simulink model "youBot_Arm_before_acceleration_test"  (R2024a)
settings: Solver=ode15s  StartTime=0.0  StopTime=3.3  MaxStep=1e-2  RelTol=1e-3  AbsTol=1e-4
model workspace: external: MATLAB File youBot_DataFile.m (data not in the file)
undefined symbols (not defined in the file): Extr_Data_LinkHoles, Qt, sigbuilder_block, smiData, X, Y, YBT_Par, Z
libraries: sm_lib x193, nesl_utility x130, fl_lib x53, simulink x13, Parts_Lib x10, MyMath_lib x8, Motor_Lib x5, Contact_Forces_Lib x4, ee_lib x2, sdl_lib x2
(part 6 of 8)

== system youBot_Arm_before_acceleration_test/Arm/Actuation/Motor/Gripper/Motor ==
  C : Inport
  Meas P : Subsystem  Tag=CustomStyle
      mask Display: disp('m')
  Motor : Motor_Lib/Motor  VariantControl=Motor  r_motor=YBT_Par.Gripper.Motor.R  l_motor=YBT_Par.Gripper.Motor.L  k_motor=1/YBT_Par.Gripper.Motor.K  i_motor_noLoad=YBT_Par.Gripper.Motor.no_load_i  v_supply=YBT_Par.Battery.v  gear_ratio=YBT_Par.Gripper.Motor.gr  friction_visc=YBT_Par.Gripper.Motor.friction  ctrl_deadZone=YBT_Par.Control.Dead_Band
  RevoluteWristGripperPivot : sm_lib/Joints/Revolute Joint  JointMode=Normal  CompositeWrenchDir=FollowerOnBase  CompositeWrenchFrame=BaseFrame  SenseConstraintForce=on  SenseConstraintTorque=off  SenseTotalForce=off  SenseTotalTorque=off  PositionTargetSpecify=on  PositionTargetPriority=Low  PositionTargetValue=smiData.RevoluteJoint(4).Rz.Pos  PositionTargetValueUnits=deg  VelocityTargetSpecify=off  VelocityTargetPriority=High  VelocityTargetValue=0  VelocityTargetValueUnits=deg/s  EquilibriumPosition=0  EquilibriumPositionUnits=rad  SpringStiffness=0  SpringStiffnessUnits=N*m/rad  DampingCoefficient=0  DampingCoefficientUnits=N*m/(rad/s)  LowerLimitSpecify=off  LowerLimitBound=-90  LowerLimitBoundUnits=deg  LowerLimitStiffness=1e4  LowerLimitStiffnessUnits=N*m/deg  LowerLimitDamping=10  LowerLimitDampingUnits=N*m/(deg/s)  LowerLimitTransitionRegionWidth=0.1  LowerLimitTransitionRegionWidthUnits=deg  UpperLimitSpecify=off  UpperLimitBound=90  UpperLimitBoundUnits=deg  UpperLimitStiffness=1e4  UpperLimitStiffnessUnits=N*m/deg  UpperLimitDamping=10  UpperLimitDampingUnits=N*m/(deg/s)  UpperLimitTransitionRegionWidth=0.1  UpperLimitTransitionRegionWidthUnits=deg  TorqueActuationMode=InputTorque  MotionActuationMode=ComputedMotion  SensePosition=on  SenseVelocity=on  SenseAcceleration=off  SenseTorqueForce=on  SenseLowerLimitTorqueForce=off  SenseUpperLimitTorqueForce=off
  Sensing i : Subsystem
      mask Display: disp('i')
  B : PMIOPort  Side=Left
  F : PMIOPort  Port=2  Side=Right
  - : PMIOPort  Port=3  Side=Right
  + : PMIOPort  Port=4  Side=Left
  m : Outport  VectorParamsAs1DForOutWhenUnconnected=off
  wires:
  Meas P/1(m) -> m/1
  C/1 -> Motor/1
  connections:
  RevoluteWristGripperPivot/RConn2 -- Motor/RConn1 -- Meas P/LConn1
  RevoluteWristGripperPivot/RConn4 -- Meas P/LConn3
  RevoluteWristGripperPivot/RConn3 -- Motor/RConn2 -- Meas P/LConn2
  RevoluteWristGripperPivot/LConn2 -- Motor/LConn1
  RevoluteWristGripperPivot/RConn1 -- F/RConn1
  RevoluteWristGripperPivot/LConn1 -- B/RConn1
  Sensing i/LConn1 -- Motor/RConn3
  Motor/LConn2 -- +/RConn1
  Sensing i/RConn2 -- -/RConn1
  Meas P/LConn5 -- Sensing i/RConn1
  RevoluteWristGripperPivot/RConn5 -- Meas P/LConn4

== system youBot_Arm_before_acceleration_test/Arm/Actuation/Motor/Pivot/Ideal ==
  C : Inport
  Current Source : fl_lib/Electrical/Electrical Sources/Controlled Current Source
  Meas P : Subsystem  Tag=CustomStyle
      mask Display: disp('m')
  PS Abs : MyMath_lib/PS Abs
      settings: InternalSimscapePortConfiguration="{\"Bottom\":[],\"Left\":[{\"id\":\"I\",\"label\":\"\",\"type\":\"input\"}],\"Right\":[{\"id\":\"O\",\"label\":\"\",\"type\":\"output\"}],\"Top\":[]}"
  PS Motor Const : fl_lib/Physical Signals/Functions/PS Gain  gain=YBT_Par.Pivot.Motor.K/YBT_Par.Pivot.Motor.gr s^2 / (kg*m^2)
  Resistor : fl_lib/Electrical/Electrical Elements/Resistor  R=YBT_Par.Pivot.Motor.R Ohm  i_specify=off  i_priority=None  i=0 A  i_nominal_specify=off  i_nominal_value=1  i_nominal_unit=A  v_specify=off  v_priority=None  v=0 V  v_nominal_specify=off  v_nominal_value=1  v_nominal_unit=V
  RevoluteBasePivot : sm_lib/Joints/Revolute Joint  JointMode=Normal  CompositeWrenchDir=FollowerOnBase  CompositeWrenchFrame=BaseFrame  SenseConstraintForce=on  SenseConstraintTorque=off  SenseTotalForce=off  SenseTotalTorque=off  PositionTargetSpecify=on  PositionTargetPriority=Low  PositionTargetValue=smiData.RevoluteJoint(3).Rz.Pos  PositionTargetValueUnits=deg  VelocityTargetSpecify=off  VelocityTargetPriority=High  VelocityTargetValue=0  VelocityTargetValueUnits=deg/s  EquilibriumPosition=0  EquilibriumPositionUnits=rad  SpringStiffness=0  SpringStiffnessUnits=N*m/rad  DampingCoefficient=YBT_Par.Pivot.Motor.friction  DampingCoefficientUnits=N*m/(rad/s)  LowerLimitSpecify=off  LowerLimitBound=-90  LowerLimitBoundUnits=deg  LowerLimitStiffness=1e4  LowerLimitStiffnessUnits=N*m/deg  LowerLimitDamping=10  LowerLimitDampingUnits=N*m/(deg/s)  LowerLimitTransitionRegionWidth=0.1  LowerLimitTransitionRegionWidthUnits=deg  UpperLimitSpecify=off  UpperLimitBound=90  UpperLimitBoundUnits=deg  UpperLimitStiffness=1e4  UpperLimitStiffnessUnits=N*m/deg  UpperLimitDamping=10  UpperLimitDampingUnits=N*m/(deg/s)  UpperLimitTransitionRegionWidth=0.1  UpperLimitTransitionRegionWidthUnits=deg  TorqueActuationMode=ComputedTorque  MotionActuationMode=InputMotion  SensePosition=on  SenseVelocity=on  SenseAcceleration=off  SenseTorqueForce=on  SenseLowerLimitTorqueForce=off  SenseUpperLimitTorqueForce=off
  Simulink-PS Converter : nesl_utility/Simulink-PS Converter  Tag=CustomStyle  PhysicalDomain=network_engine_domain  SubClassName=ps_input  LeftPortType=input  RightPortType=output  PseudoPeriodic=off  Frequencies=[]  NoiseDistribution=none  NoiseParameters=[]  Unit=deg  AffineConversion=off  FilteringAndDerivatives=filter  SimscapeFilterOrder=2  InputFilterTimeConstant=0.005  UdotUserProvided=1
  B : PMIOPort  Side=Left
  F : PMIOPort  Port=2  Side=Right
  + : PMIOPort  Port=3  Side=Left
  - : PMIOPort  Port=4  Side=Right
  m : Outport  VectorParamsAs1DForOutWhenUnconnected=off
  wires:
  Meas P/1(P) -> m/1
  C/1 -> Simulink-PS Converter/1
  connections:
  Resistor/RConn1 -- -/RConn1
  PS Abs/RConn1 -- Meas P/LConn5 -- Current Source/RConn1
  RevoluteBasePivot/RConn2 -- Meas P/LConn1
  RevoluteBasePivot/RConn4 -- PS Motor Const/LConn1 -- Meas P/LConn3
  RevoluteBasePivot/RConn3 -- Meas P/LConn2
  Resistor/LConn1 -- Current Source/LConn1
  +/RConn1 -- Current Source/RConn2
  PS Motor Const/RConn1 -- PS Abs/LConn1
  RevoluteBasePivot/LConn2 -- Simulink-PS Converter/RConn1
  RevoluteBasePivot/RConn1 -- F/RConn1
  RevoluteBasePivot/LConn1 -- B/RConn1
  RevoluteBasePivot/RConn5 -- Meas P/LConn4

== system youBot_Arm_before_acceleration_test/Arm/Actuation/Motor/Pivot/Motor ==
  C : Inport
  Meas P : Subsystem  Tag=CustomStyle
      mask Display: disp('m')
  Motor : Motor_Lib/Motor  VariantControl=Motor  r_motor=YBT_Par.Pivot.Motor.R  l_motor=YBT_Par.Pivot.Motor.L  k_motor=1/YBT_Par.Pivot.Motor.K  i_motor_noLoad=YBT_Par.Pivot.Motor.no_load_i  v_supply=YBT_Par.Battery.v  gear_ratio=YBT_Par.Pivot.Motor.gr  friction_visc=YBT_Par.Pivot.Motor.friction  ctrl_deadZone=YBT_Par.Control.Dead_Band
  RevolutePivotBicep : sm_lib/Joints/Revolute Joint  JointMode=Normal  CompositeWrenchDir=FollowerOnBase  CompositeWrenchFrame=BaseFrame  SenseConstraintForce=on  SenseConstraintTorque=off  SenseTotalForce=off  SenseTotalTorque=off  PositionTargetSpecify=on  PositionTargetPriority=Low  PositionTargetValue=smiData.RevoluteJoint(1).Rz.Pos  PositionTargetValueUnits=deg  VelocityTargetSpecify=off  VelocityTargetPriority=High  VelocityTargetValue=0  VelocityTargetValueUnits=deg/s  EquilibriumPosition=0  EquilibriumPositionUnits=rad  SpringStiffness=0  SpringStiffnessUnits=N*m/rad  DampingCoefficient=YBT_Par.Bicep.Motor.friction*0  DampingCoefficientUnits=N*m/(rad/s)  LowerLimitSpecify=off  LowerLimitBound=-90  LowerLimitBoundUnits=deg  LowerLimitStiffness=1e4  LowerLimitStiffnessUnits=N*m/deg  LowerLimitDamping=10  LowerLimitDampingUnits=N*m/(deg/s)  LowerLimitTransitionRegionWidth=0.1  LowerLimitTransitionRegionWidthUnits=deg  UpperLimitSpecify=off  UpperLimitBound=90  UpperLimitBoundUnits=deg  UpperLimitStiffness=1e4  UpperLimitStiffnessUnits=N*m/deg  UpperLimitDamping=10  UpperLimitDampingUnits=N*m/(deg/s)  UpperLimitTransitionRegionWidth=0.1  UpperLimitTransitionRegionWidthUnits=deg  TorqueActuationMode=InputTorque  MotionActuationMode=ComputedMotion  SensePosition=on  SenseVelocity=on  SenseAcceleration=off  SenseTorqueForce=on  SenseLowerLimitTorqueForce=off  SenseUpperLimitTorqueForce=off
  Sensing i : Subsystem
      mask Display: disp('i')
  B : PMIOPort  Side=Left
  F : PMIOPort  Port=2  Side=Right
  - : PMIOPort  Port=3  Side=Right
  + : PMIOPort  Port=4  Side=Left
  m : Outport  VectorParamsAs1DForOutWhenUnconnected=off
  wires:
  Meas P/1(P) -> m/1
  C/1 -> Motor/1
  connections:
  RevolutePivotBicep/RConn2 -- Meas P/LConn1 -- Motor/RConn1
  Meas P/LConn3 -- RevolutePivotBicep/RConn4
  RevolutePivotBicep/RConn3 -- Meas P/LConn2 -- Motor/RConn2
  Motor/LConn1 -- RevolutePivotBicep/LConn2
  RevolutePivotBicep/RConn1 -- F/RConn1
  RevolutePivotBicep/LConn1 -- B/RConn1
  Sensing i/LConn1 -- Motor/RConn3
  Motor/LConn2 -- +/RConn1
  Sensing i/RConn2 -- -/RConn1
  Sensing i/RConn1 -- Meas P/LConn5
  RevolutePivotBicep/RConn5 -- Meas P/LConn4

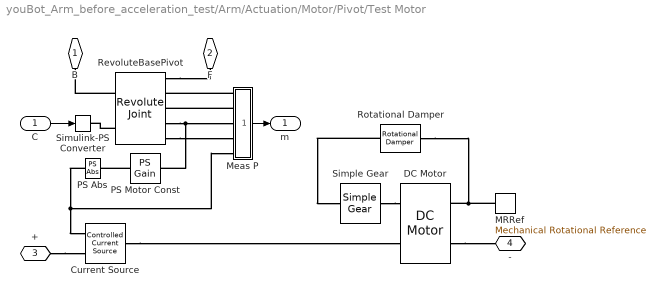
== system youBot_Arm_before_acceleration_test/Arm/Actuation/Motor/Pivot/Test Motor ==
  C : Inport
  Current Source : fl_lib/Electrical/Electrical Sources/Controlled Current Source
  DC Motor : ee_lib/Electromechanical/Brushed Motors/DC Motor  field_option=ee.enum.field_option.pm  Rf=100 Ohm  Lf=1 H  Laf=0.15 H  If0=0 A  parameterization=1  Ra=YBT_Par.Pivot.Motor.R Ohm  La=YBT_Par.Pivot.Motor.L H  emf_or_torque=2  Kv=YBT_Par.Pivot.Motor.K V/rpm  Ki=1/YBT_Par.Pivot.Motor.K N*m/A  T_stall=2.4e-4 N*m  w_max=1.91e+4 rpm  w_rated=1.5e+4 rpm  P_rated=0.08 W  V_rated=1.5 V  lam_param=2  i_noload=YBT_Par.Pivot.Motor.no_load_i A  V_i_noload=24 V  J=0 g*cm^2  lam=0 N*m/(rad/s)  speed0=0 rpm  enable_fault_armature=simscape.enum.onoff.off  rev_faulted=1 / 3  G_faulted_armature=1e-5 S  fault_trigger_armature=ee.enum.faults.faultTrigger.temporal  t_fault_armature=1 s  max_permissible_current_armature=inf A  t_fail_on_current_armature=1 s  enable_fault_field=simscape.enum.onoff.off  G_faulted_field=1e-5 S  fault_trigger_field=ee.enum.faults.faultTrigger.temporal  t_fault_field=1 s  max_permissible_current_field=inf A  t_fail_on_current_field=1 s  fault_action=simscape.enum.assert.action.none  alpha=3.93e-3 1/K  Tmeas=25 degC  thermal_mass=100 J/K  initial_temperature=25 degC
  MRRef : fl_lib/Mechanical/Rotational Elements/Mechanical Rotational Reference
  Meas P : Subsystem  Tag=CustomStyle
      mask Display: disp('m')
  PS Abs : MyMath_lib/PS Abs
      settings: InternalSimscapePortConfiguration="{\"Bottom\":[],\"Left\":[{\"id\":\"I\",\"label\":\"\",\"type\":\"input\"}],\"Right\":[{\"id\":\"O\",\"label\":\"\",\"type\":\"output\"}],\"Top\":[]}"
  PS Motor Const : fl_lib/Physical Signals/Functions/PS Gain  gain=YBT_Par.Pivot.Motor.K/YBT_Par.Pivot.Motor.gr s^2 / (kg*m^2)
  RevoluteBasePivot : sm_lib/Joints/Revolute Joint  JointMode=Normal  CompositeWrenchDir=FollowerOnBase  CompositeWrenchFrame=BaseFrame  SenseConstraintForce=on  SenseConstraintTorque=off  SenseTotalForce=off  SenseTotalTorque=off  PositionTargetSpecify=on  PositionTargetPriority=Low  PositionTargetValue=smiData.RevoluteJoint(3).Rz.Pos  PositionTargetValueUnits=deg  VelocityTargetSpecify=off  VelocityTargetPriority=High  VelocityTargetValue=0  VelocityTargetValueUnits=deg/s  EquilibriumPosition=0  EquilibriumPositionUnits=rad  SpringStiffness=0  SpringStiffnessUnits=N*m/rad  DampingCoefficient=0  DampingCoefficientUnits=N*m/(rad/s)  LowerLimitSpecify=off  LowerLimitBound=-90  LowerLimitBoundUnits=deg  LowerLimitStiffness=1e4  LowerLimitStiffnessUnits=N*m/deg  LowerLimitDamping=10  LowerLimitDampingUnits=N*m/(deg/s)  LowerLimitTransitionRegionWidth=0.1  LowerLimitTransitionRegionWidthUnits=deg  UpperLimitSpecify=off  UpperLimitBound=90  UpperLimitBoundUnits=deg  UpperLimitStiffness=1e4  UpperLimitStiffnessUnits=N*m/deg  UpperLimitDamping=10  UpperLimitDampingUnits=N*m/(deg/s)  UpperLimitTransitionRegionWidth=0.1  UpperLimitTransitionRegionWidthUnits=deg  TorqueActuationMode=ComputedTorque  MotionActuationMode=InputMotion  SensePosition=on  SenseVelocity=on  SenseAcceleration=off  SenseTorqueForce=on  SenseLowerLimitTorqueForce=off  SenseUpperLimitTorqueForce=off
  Rotational Damper : fl_lib/Mechanical/Rotational Elements/Rotational Damper  D=0.001 N*m/(rad/s)  w_specify=off  w_priority=None  w=0 rad/s  w_nominal_specify=off  w_nominal_value=1  w_nominal_unit=rad/s  t_specify=off  t_priority=None  t=0 N*m  t_nominal_specify=off  t_nominal_value=1  t_nominal_unit=N*m
  Simple Gear : sdl_lib/Gears/Simple Gear  ratio=YBT_Par.Pivot.Motor.gr  rotation_direction=3-2*(1)  enable_faults=simscape.enum.onoff.off  efficiency_fault=0.05  fault_angles=pi / 12 rad  friction_model=1  T_noload=0.1 N*m  T_nom=5 N*m  efficiency_nom=0.8  efficiency=0.8  temperature_TLU=[ 280 300 320 ] K  load_TLU=[ 1 5 10 ] N*m  efficiency_TLU=[ 0.95 0.9 0.85 ]  efficiency_TLU2=[ 0.85 0.8 0.75; 0.95 0.9 0.85; 0.85 0.8 0.7 ]  w_thr=0.01 rad/s  pwr_thr=0.001 W  enable_backlash=false  hardstop_model=simscape.enum.hardstop.smooth  backlash_distance=1e-3 mm  r_base=0.1 m  transition=1e-4 mm  backlash_stiffness=1e7 N/m  backlash_damping=1e6 N*s/m  coeff_rest=0  v_tol=0.001 m/s  f_tol=0 N  mu_visc=[ 0 0 ] N*m/(rad/s)  thermal_mass=50 J/K  temperature_specify=off  temperature_priority=High  temperature=300 K  temperature_nominal_specify=off  temperature_nominal_value=1  temperature_nominal_unit=K  x_backlash_specify=off  x_backlash_priority=None  x_backlash=0 mm  x_backlash_nominal_specify=off  x_backlash_nominal_value=1  x_backlash_nominal_unit=mm  f_hardstop_specify=off  f_hardstop_priority=None  f_hardstop=0 N  f_hardstop_nominal_specify=off  f_hardstop_nominal_value=1  f_hardstop_nominal_unit=N  v_backlash_specify=off  v_backlash_priority=None  v_backlash=0 m/s  v_backlash_nominal_specify=off  v_backlash_nominal_value=1  v_backlash_nominal_unit=m/s
  Simulink-PS Converter : nesl_utility/Simulink-PS Converter  Tag=CustomStyle  PhysicalDomain=network_engine_domain  SubClassName=ps_input  LeftPortType=input  RightPortType=output  PseudoPeriodic=off  Frequencies=[]  NoiseDistribution=none  NoiseParameters=[]  Unit=deg  AffineConversion=off  FilteringAndDerivatives=filter  SimscapeFilterOrder=2  InputFilterTimeConstant=0.005  UdotUserProvided=1
  B : PMIOPort  Side=Left
  F : PMIOPort  Port=2  Side=Right
  + : PMIOPort  Port=3  Side=Left
  - : PMIOPort  Port=4  Side=Right
  m : Outport  VectorParamsAs1DForOutWhenUnconnected=off
  wires:
  C/1 -> Simulink-PS Converter/1
  Meas P/1(P) -> m/1
  connections:
  RevoluteBasePivot/LConn1 -- B/RConn1
  RevoluteBasePivot/RConn1 -- F/RConn1
  RevoluteBasePivot/LConn2 -- Simulink-PS Converter/RConn1
  PS Motor Const/RConn1 -- PS Abs/LConn1
  +/RConn1 -- Current Source/RConn2
  Current Source/LConn1 -- DC Motor/LConn1
  Meas P/LConn2 -- RevoluteBasePivot/RConn3
  RevoluteBasePivot/RConn4 -- PS Motor Const/LConn1 -- Meas P/LConn3
  Meas P/LConn1 -- RevoluteBasePivot/RConn2
  PS Abs/RConn1 -- Meas P/LConn5 -- Current Source/RConn1
  DC Motor/RConn1 -- -/RConn1
  MRRef/LConn1 -- Rotational Damper/RConn1 -- DC Motor/RConn2
  Simple Gear/LConn1 -- DC Motor/LConn2
  Rotational Damper/LConn1 -- Simple Gear/RConn1
  RevoluteBasePivot/RConn5 -- Meas P/LConn4

== system youBot_Arm_before_acceleration_test/Arm/Actuation/Motor/Wrist/Ideal ==
  C : Inport
  Current Source : fl_lib/Electrical/Electrical Sources/Controlled Current Source
  Meas W : Subsystem
      mask Display: disp('m')
  PS Abs : MyMath_lib/PS Abs
      settings: InternalSimscapePortConfiguration="{\"Bottom\":[],\"Left\":[{\"id\":\"I\",\"label\":\"\",\"type\":\"input\"}],\"Right\":[{\"id\":\"O\",\"label\":\"\",\"type\":\"output\"}],\"Top\":[]}"
  PS Motor Const : fl_lib/Physical Signals/Functions/PS Gain  gain=YBT_Par.Wrist.Motor.K/YBT_Par.Wrist.Motor.gr s^2 / (kg*m^2)
  Resistor : fl_lib/Electrical/Electrical Elements/Resistor  R=YBT_Par.Wrist.Motor.R Ohm  i_specify=off  i_priority=None  i=0 A  i_nominal_specify=off  i_nominal_value=1  i_nominal_unit=A  v_specify=off  v_priority=None  v=0 V  v_nominal_specify=off  v_nominal_value=1  v_nominal_unit=V
  RevoluteForearmWrist : sm_lib/Joints/Revolute Joint  JointMode=Normal  CompositeWrenchDir=FollowerOnBase  CompositeWrenchFrame=BaseFrame  SenseConstraintForce=on  SenseConstraintTorque=off  SenseTotalForce=off  SenseTotalTorque=off  PositionTargetSpecify=on  PositionTargetPriority=Low  PositionTargetValue=smiData.RevoluteJoint(5).Rz.Pos  PositionTargetValueUnits=deg  VelocityTargetSpecify=off  VelocityTargetPriority=High  VelocityTargetValue=0  VelocityTargetValueUnits=deg/s  EquilibriumPosition=0  EquilibriumPositionUnits=rad  SpringStiffness=0  SpringStiffnessUnits=N*m/rad  DampingCoefficient=YBT_Par.Wrist.Motor.friction  DampingCoefficientUnits=N*m/(rad/s)  LowerLimitSpecify=off  LowerLimitBound=-90  LowerLimitBoundUnits=deg  LowerLimitStiffness=1e4  LowerLimitStiffnessUnits=N*m/deg  LowerLimitDamping=10  LowerLimitDampingUnits=N*m/(deg/s)  LowerLimitTransitionRegionWidth=0.1  LowerLimitTransitionRegionWidthUnits=deg  UpperLimitSpecify=off  UpperLimitBound=90  UpperLimitBoundUnits=deg  UpperLimitStiffness=1e4  UpperLimitStiffnessUnits=N*m/deg  UpperLimitDamping=10  UpperLimitDampingUnits=N*m/(deg/s)  UpperLimitTransitionRegionWidth=0.1  UpperLimitTransitionRegionWidthUnits=deg  TorqueActuationMode=ComputedTorque  MotionActuationMode=InputMotion  SensePosition=on  SenseVelocity=on  SenseAcceleration=off  SenseTorqueForce=on  SenseLowerLimitTorqueForce=off  SenseUpperLimitTorqueForce=off
  Simulink-PS Converter5 : nesl_utility/Simulink-PS Converter  Tag=CustomStyle  PhysicalDomain=network_engine_domain  SubClassName=ps_input  LeftPortType=input  RightPortType=output  PseudoPeriodic=off  Frequencies=[]  NoiseDistribution=none  NoiseParameters=[]  Unit=deg  AffineConversion=off  FilteringAndDerivatives=filter  SimscapeFilterOrder=2  InputFilterTimeConstant=0.005  UdotUserProvided=1
  B : PMIOPort  Side=Left
  F : PMIOPort  Port=2  Side=Right
  + : PMIOPort  Port=3  Side=Left
  - : PMIOPort  Port=4  Side=Right
  m : Outport  VectorParamsAs1DForOutWhenUnconnected=off
  wires:
  C/1 -> Simulink-PS Converter5/1
  Meas W/1(W) -> m/1
  connections:
  PS Abs/RConn1 -- Meas W/LConn5 -- Current Source/RConn1
  PS Motor Const/RConn1 -- PS Abs/LConn1
  -/RConn1 -- Resistor/RConn1
  Resistor/LConn1 -- Current Source/LConn1
  RevoluteForearmWrist/LConn2 -- Simulink-PS Converter5/RConn1
  Meas W/LConn3 -- PS Motor Const/LConn1 -- RevoluteForearmWrist/RConn4
  RevoluteForearmWrist/RConn2 -- Meas W/LConn1
  RevoluteForearmWrist/RConn3 -- Meas W/LConn2
  Current Source/RConn2 -- +/RConn1
  RevoluteForearmWrist/RConn1 -- F/RConn1
  RevoluteForearmWrist/LConn1 -- B/RConn1
  RevoluteForearmWrist/RConn5 -- Meas W/LConn4

== system youBot_Arm_before_acceleration_test/Arm/Actuation/Motor/Wrist/Motor ==
  C : Inport
  Meas P : Subsystem  Tag=CustomStyle
      mask Display: disp('m')
  Motor : Motor_Lib/Motor  VariantControl=Motor  r_motor=YBT_Par.Wrist.Motor.R  l_motor=YBT_Par.Wrist.Motor.L  k_motor=1/YBT_Par.Wrist.Motor.K  i_motor_noLoad=YBT_Par.Wrist.Motor.no_load_i  v_supply=YBT_Par.Battery.v  gear_ratio=YBT_Par.Wrist.Motor.gr  friction_visc=YBT_Par.Wrist.Motor.friction  ctrl_deadZone=YBT_Par.Control.Dead_Band
  RevoluteForearmWrist : sm_lib/Joints/Revolute Joint  JointMode=Normal  CompositeWrenchDir=FollowerOnBase  CompositeWrenchFrame=BaseFrame  SenseConstraintForce=on  SenseConstraintTorque=off  SenseTotalForce=off  SenseTotalTorque=off  PositionTargetSpecify=on  PositionTargetPriority=Low  PositionTargetValue=smiData.RevoluteJoint(5).Rz.Pos  PositionTargetValueUnits=deg  VelocityTargetSpecify=off  VelocityTargetPriority=High  VelocityTargetValue=0  VelocityTargetValueUnits=deg/s  EquilibriumPosition=0  EquilibriumPositionUnits=rad  SpringStiffness=0  SpringStiffnessUnits=N*m/rad  DampingCoefficient=0  DampingCoefficientUnits=N*m/(rad/s)  LowerLimitSpecify=off  LowerLimitBound=-90  LowerLimitBoundUnits=deg  LowerLimitStiffness=1e4  LowerLimitStiffnessUnits=N*m/deg  LowerLimitDamping=10  LowerLimitDampingUnits=N*m/(deg/s)  LowerLimitTransitionRegionWidth=0.1  LowerLimitTransitionRegionWidthUnits=deg  UpperLimitSpecify=off  UpperLimitBound=90  UpperLimitBoundUnits=deg  UpperLimitStiffness=1e4  UpperLimitStiffnessUnits=N*m/deg  UpperLimitDamping=10  UpperLimitDampingUnits=N*m/(deg/s)  UpperLimitTransitionRegionWidth=0.1  UpperLimitTransitionRegionWidthUnits=deg  TorqueActuationMode=InputTorque  MotionActuationMode=ComputedMotion  SensePosition=on  SenseVelocity=on  SenseAcceleration=off  SenseTorqueForce=on  SenseLowerLimitTorqueForce=off  SenseUpperLimitTorqueForce=off
  Sensing i : Subsystem
      mask Display: disp('i')
  B : PMIOPort  Side=Left
  F : PMIOPort  Port=2  Side=Right
  - : PMIOPort  Port=3  Side=Right
  + : PMIOPort  Port=4  Side=Left
  m : Outport  VectorParamsAs1DForOutWhenUnconnected=off
  wires:
  Meas P/1(m) -> m/1
  C/1 -> Motor/1
  connections:
  RevoluteForearmWrist/RConn2 -- Motor/RConn1 -- Meas P/LConn1
  RevoluteForearmWrist/RConn4 -- Meas P/LConn3
  RevoluteForearmWrist/RConn3 -- Motor/RConn2 -- Meas P/LConn2
  RevoluteForearmWrist/LConn2 -- Motor/LConn1
  RevoluteForearmWrist/RConn1 -- F/RConn1
  RevoluteForearmWrist/LConn1 -- B/RConn1
  Sensing i/LConn1 -- Motor/RConn3
  Motor/LConn2 -- +/RConn1
  Sensing i/RConn2 -- -/RConn1
  Meas P/LConn5 -- Sensing i/RConn1
  RevoluteForearmWrist/RConn5 -- Meas P/LConn4

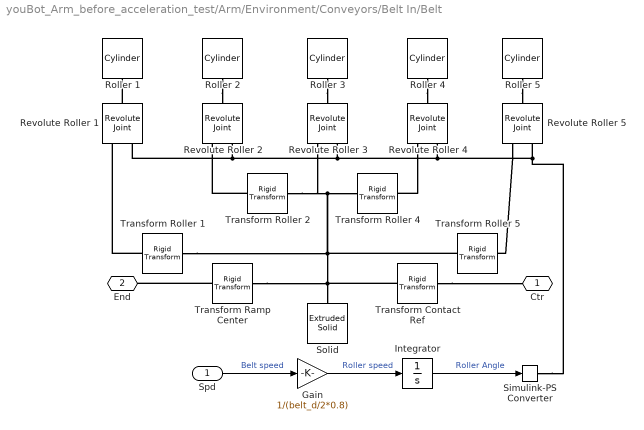
== system youBot_Arm_before_acceleration_test/Arm/Environment/Conveyors/Belt In/Belt ==
  Spd : Inport
  Gain : Gain  Gain=1/(belt_d/2*0.8)
  Integrator : Integrator
  Revolute Roller {1..5} (5 alike) : sm_lib/Joints/Revolute Joint  JointMode=Normal  CompositeWrenchDir=FollowerOnBase  CompositeWrenchFrame=BaseFrame  SenseConstraintForce=off  SenseConstraintTorque=off  SenseTotalForce=off  SenseTotalTorque=off  PositionTargetSpecify=off  PositionTargetPriority=High  PositionTargetValue=0  PositionTargetValueUnits=deg  VelocityTargetSpecify=off  VelocityTargetPriority=High  VelocityTargetValue=0  VelocityTargetValueUnits=deg/s  EquilibriumPosition=0  EquilibriumPositionUnits=deg  SpringStiffness=0  SpringStiffnessUnits=N*m/deg  DampingCoefficient=0  DampingCoefficientUnits=N*m/(deg/s)  LowerLimitSpecify=off  LowerLimitBound=-90  LowerLimitBoundUnits=deg  LowerLimitStiffness=1e4  LowerLimitStiffnessUnits=N*m/deg  LowerLimitDamping=10  LowerLimitDampingUnits=N*m/(deg/s)  LowerLimitTransitionRegionWidth=0.1  LowerLimitTransitionRegionWidthUnits=deg  UpperLimitSpecify=off  UpperLimitBound=90  UpperLimitBoundUnits=deg  UpperLimitStiffness=1e4  UpperLimitStiffnessUnits=N*m/deg  UpperLimitDamping=10  UpperLimitDampingUnits=N*m/(deg/s)  UpperLimitTransitionRegionWidth=0.1  UpperLimitTransitionRegionWidthUnits=deg  TorqueActuationMode=ComputedTorque  MotionActuationMode=InputMotion  SensePosition=off  SenseVelocity=off  SenseAcceleration=off  SenseTorqueForce=off  SenseLowerLimitTorqueForce=off  SenseUpperLimitTorqueForce=off
  Roller {1..5} (5 alike) : Parts_Lib/Cylinder  Tag=CustomStyle  cyl_radius=belt_d/2*0.8  cyl_length=belt_w  cyl_density=1000  cyl_color=custom  cyl_opacity=1  cyl_color_custom=roller_clr  mark_radius=[0.75 0.5]  mark_len_factor=1.01  mark_angle=60  mark_color=black  mark_opacity=1
  Simulink-PS Converter : nesl_utility/Simulink-PS Converter  PhysicalDomain=network_engine_domain  SubClassName=ps_input  LeftPortType=input  RightPortType=output  PseudoPeriodic=off  Frequencies=[]  NoiseDistribution=none  NoiseParameters=[]  Unit=1  AffineConversion=off  FilteringAndDerivatives=filter  SimscapeFilterOrder=2  InputFilterTimeConstant=0.005  UdotUserProvided=1
  Solid : sm_lib/Body Elements/Extruded Solid  ExtrusionType=General  PolygonNumSides=3  PolygonOuterRadius=1  PolygonOuterRadiusUnits=m  ExportEntireGeometry=off  ExtrusionCrossSection=Extr_Data_LinkHoles(belt_l,belt_d,0.8*belt_d/2,5)  ExtrusionCrossSectionUnits=m  ExportConvexHullGeometry=off  ExtrusionLength=belt_w  ExtrusionLengthUnits=m  InertiaType=CalculateFromGeometry  BasedOnType=Density  Density=1000  DensityUnits=kg/(m^3)  Mass=1  MassUnits=kg  CenterOfMass=[0 0 0]  CenterOfMassUnits=m  MomentsOfInertia=[1 1 1]  MomentsOfInertiaUnits=kg*m^2  ProductsOfInertia=[0 0 0]  ProductsOfInertiaUnits=kg*m^2  GraphicType=FromGeometry  MarkerShape=Sphere  MarkerSize=10  GraphicVisPropType=SimpleVisualProperties  GraphicDiffuseColor=[0.5 0.5 0.5]  GraphicOpacity=1.0  GraphicSpecularColor=[0.5 0.5 0.5 1.0]  GraphicAmbientColor=[0.15 0.15 0.15 1.0]  GraphicEmissiveColor=[0.0 0.0 0.0 1.0]  GraphicShininess=75  DoExposeReferenceFrame=on  SerializedFrames=<Frames/>
  Transform Contact Ref : sm_lib/Frames and Transforms/Rigid Transform  RotationMethod=RotationSequence  FollAlignAxisA=+X  BaseAlignAxisA=+Y  FollAlignAxisB=+Y  BaseAlignAxisB=+Z  RotationStandardAxis=+Z  RotationAngle=0  RotationAngleUnits=deg  RotationArbitraryAxis=[0 0 1]  RotationSequenceAxes=FollowerAxes  RotationSequence=XYZ  RotationSequenceAngles=[-90 0 0]  RotationSequenceAnglesUnits=deg  RotationMatrix=[1 0 0; 0 1 0; 0 0 1]  Quaternion=[1 0 0 0]  TranslationMethod=None  TranslationCartesianOffset=[0 0 0]  TranslationCartesianOffsetUnits=m  TranslationStandardAxis=+X  TranslationStandardOffset=3/2  TranslationStandardOffsetUnits=m  TranslationROffset=0  TranslationROffsetUnits=m  TranslationThetaOffset=0  TranslationThetaOffsetUnits=deg  TranslationZOffset=0  TranslationZOffsetUnits=m
  Transform Ramp Center : sm_lib/Frames and Transforms/Rigid Transform  RotationMethod=None  FollAlignAxisA=+X  BaseAlignAxisA=+Y  FollAlignAxisB=+Y  BaseAlignAxisB=+Z  RotationStandardAxis=+Z  RotationAngle=0  RotationAngleUnits=deg  RotationArbitraryAxis=[0 0 1]  RotationSequenceAxes=FollowerAxes  RotationSequence=XYX  RotationSequenceAngles=[0 0 0]  RotationSequenceAnglesUnits=deg  RotationMatrix=[1 0 0; 0 1 0; 0 0 1]  Quaternion=[1 0 0 0]  TranslationMethod=StandardAxis  TranslationCartesianOffset=[0 0 0]  TranslationCartesianOffsetUnits=m  TranslationStandardAxis=+X  TranslationStandardOffset=belt_l/2  TranslationStandardOffsetUnits=m  TranslationROffset=0  TranslationROffsetUnits=m  TranslationThetaOffset=0  TranslationThetaOffsetUnits=deg  TranslationZOffset=0  TranslationZOffsetUnits=m
  Transform Roller 1 : sm_lib/Frames and Transforms/Rigid Transform  RotationMethod=None  FollAlignAxisA=+X  BaseAlignAxisA=+Y  FollAlignAxisB=+Y  BaseAlignAxisB=+Z  RotationStandardAxis=+Z  RotationAngle=0  RotationAngleUnits=deg  RotationArbitraryAxis=[0 0 1]  RotationSequenceAxes=FollowerAxes  RotationSequence=XYX  RotationSequenceAngles=[0 0 0]  RotationSequenceAnglesUnits=deg  RotationMatrix=[1 0 0; 0 1 0; 0 0 1]  Quaternion=[1 0 0 0]  TranslationMethod=StandardAxis  TranslationCartesianOffset=[0 0 0]  TranslationCartesianOffsetUnits=m  TranslationStandardAxis=-X  TranslationStandardOffset=belt_l/2  TranslationStandardOffsetUnits=m  TranslationROffset=0  TranslationROffsetUnits=m  TranslationThetaOffset=0  TranslationThetaOffsetUnits=deg  TranslationZOffset=0  TranslationZOffsetUnits=m
  Transform Roller 2 : sm_lib/Frames and Transforms/Rigid Transform  RotationMethod=None  FollAlignAxisA=+X  BaseAlignAxisA=+Y  FollAlignAxisB=+Y  BaseAlignAxisB=+Z  RotationStandardAxis=+Z  RotationAngle=0  RotationAngleUnits=deg  RotationArbitraryAxis=[0 0 1]  RotationSequenceAxes=FollowerAxes  RotationSequence=XYX  RotationSequenceAngles=[0 0 0]  RotationSequenceAnglesUnits=deg  RotationMatrix=[1 0 0; 0 1 0; 0 0 1]  Quaternion=[1 0 0 0]  TranslationMethod=StandardAxis  TranslationCartesianOffset=[0 0 0]  TranslationCartesianOffsetUnits=m  TranslationStandardAxis=-X  TranslationStandardOffset=belt_l/4  TranslationStandardOffsetUnits=m  TranslationROffset=0  TranslationROffsetUnits=m  TranslationThetaOffset=0  TranslationThetaOffsetUnits=deg  TranslationZOffset=0  TranslationZOffsetUnits=m
  Transform Roller 4 : sm_lib/Frames and Transforms/Rigid Transform  RotationMethod=None  FollAlignAxisA=+X  BaseAlignAxisA=+Y  FollAlignAxisB=+Y  BaseAlignAxisB=+Z  RotationStandardAxis=+Z  RotationAngle=0  RotationAngleUnits=deg  RotationArbitraryAxis=[0 0 1]  RotationSequenceAxes=FollowerAxes  RotationSequence=XYX  RotationSequenceAngles=[0 0 0]  RotationSequenceAnglesUnits=deg  RotationMatrix=[1 0 0; 0 1 0; 0 0 1]  Quaternion=[1 0 0 0]  TranslationMethod=StandardAxis  TranslationCartesianOffset=[0 0 0]  TranslationCartesianOffsetUnits=m  TranslationStandardAxis=+X  TranslationStandardOffset=belt_l/4  TranslationStandardOffsetUnits=m  TranslationROffset=0  TranslationROffsetUnits=m  TranslationThetaOffset=0  TranslationThetaOffsetUnits=deg  TranslationZOffset=0  TranslationZOffsetUnits=m
  Transform Roller 5 : sm_lib/Frames and Transforms/Rigid Transform  RotationMethod=None  FollAlignAxisA=+X  BaseAlignAxisA=+Y  FollAlignAxisB=+Y  BaseAlignAxisB=+Z  RotationStandardAxis=+Z  RotationAngle=0  RotationAngleUnits=deg  RotationArbitraryAxis=[0 0 1]  RotationSequenceAxes=FollowerAxes  RotationSequence=XYX  RotationSequenceAngles=[0 0 0]  RotationSequenceAnglesUnits=deg  RotationMatrix=[1 0 0; 0 1 0; 0 0 1]  Quaternion=[1 0 0 0]  TranslationMethod=StandardAxis  TranslationCartesianOffset=[0 0 0]  TranslationCartesianOffsetUnits=m  TranslationStandardAxis=+X  TranslationStandardOffset=belt_l/2  TranslationStandardOffsetUnits=m  TranslationROffset=0  TranslationROffsetUnits=m  TranslationThetaOffset=0  TranslationThetaOffsetUnits=deg  TranslationZOffset=0  TranslationZOffsetUnits=m
  Ctr : PMIOPort  Side=Right
  End : PMIOPort  Port=2  Side=Left
  wires:
  Integrator/1 -> Simulink-PS Converter/1  "Roller Angle"
  Gain/1 -> Integrator/1  "Roller speed"
  Spd/1 -> Gain/1  "Belt speed"
  connections:
  Revolute Roller 5/LConn2 -- Revolute Roller 4/LConn2 -- Revolute Roller 3/LConn2 -- Revolute Roller 2/LConn2 -- Revolute Roller 1/LConn2 -- Simulink-PS Converter/RConn1
  Roller 5/LConn1 -- Revolute Roller 5/RConn1
  Roller 4/LConn1 -- Revolute Roller 4/RConn1
  Roller 3/LConn1 -- Revolute Roller 3/RConn1
  Roller 2/LConn1 -- Revolute Roller 2/RConn1
  Transform Roller 1/RConn1 -- Revolute Roller 1/LConn1
  Revolute Roller 5/LConn1 -- Transform Roller 5/RConn1
  Revolute Roller 4/LConn1 -- Transform Roller 4/RConn1
  Transform Roller 2/RConn1 -- Revolute Roller 2/LConn1
  Revolute Roller 1/RConn1 -- Roller 1/LConn1
  Transform Ramp Center/LConn1 -- End/RConn1
  Transform Contact Ref/RConn1 -- Transform Ramp Center/RConn1 -- Transform Roller 5/LConn1 -- Transform Roller 1/LConn1 -- Transform Roller 4/LConn1 -- Transform Roller 2/LConn1 -- Revolute Roller 3/LConn1 -- Solid/RConn1
  Transform Contact Ref/LConn1 -- Ctr/RConn1

== system youBot_Arm_before_acceleration_test/Arm/Environment/Conveyors/Belt In/Create Bus ==
  vx : Inport
  Bus Creator : BusCreator  Inputs=3
  Enable : Constant
  vy : Constant  Value=0
  bus : Outport  VectorParamsAs1DForOutWhenUnconnected=off
  wires:
  Enable/1 -> Bus Creator/1  "Enable"
  vy/1 -> Bus Creator/3  "vy"
  vx/1 -> Bus Creator/2
  Bus Creator/1 -> bus/1

== system youBot_Arm_before_acceleration_test/Arm/Environment/Conveyors/Belt In/Detect Box ==
  Fn : Inport
  1/duration : Gain  Gain=1/dur_presence
  Check Weight : simulink/Logic and Bit Operations/Compare To Constant  relop=>=  const=box_weight  OutDataTypeStr=boolean  ZeroCross=off
  Compare To Zero : simulink/Logic and Bit Operations/Compare To Zero  relop=<=  OutDataTypeStr=boolean  ZeroCross=off
  Data Type Conversion : DataTypeConversion  OutDataTypeStr=double  SaturateOnIntegerOverflow=off  RndMeth=Floor
  Integrator : Integrator  ExternalReset=either
  Limit Level : Saturate  UpperLimit=box_weight  LowerLimit=0  ZeroCross=off
  Max Force : Saturate  UpperLimit=box_weight  LowerLimit=0
  Scope : Scope  NumInputPorts=2
  Unit Delay : UnitDelay  SampleTime=0.1  HasFrameUpgradeWarning=on
  On : Outport  VectorParamsAs1DForOutWhenUnconnected=off
  wires:
  Fn/1 -> Max Force/1
  Max Force/1 -> 1/duration/1
  Integrator/1 -> Limit Level/1
  Limit Level/1 -> Check Weight/1
  Compare To Zero/1 -> Integrator/2
  Check Weight/1 -> Data Type Conversion/1, Scope/2  "Enable Belt"
  Data Type Conversion/1 -> Unit Delay/1
  Unit Delay/1 -> On/1
  1/duration/1 -> Scope/1, Compare To Zero/1, Integrator/1

== system youBot_Arm_before_acceleration_test/Arm/Environment/Conveyors/Belt In/Light Curtain ==
  Geometry : Subsystem  mask{beam_length=YBT_Par.BeltIn.Sensor.Beam.length, beam_radius=YBT_Par.BeltIn.Sensor.Beam.radius, beam_offset=YBT_Par.BeltIn.Sensor.Beam.offset, beam_color=YBT_Par.BeltIn.Sensor.Beam.color, beam_opc=YBT_Par.BeltIn.Sensor.Beam.opacity}
      mask prompts: beam_length "Length (m)"; beam_radius "Radius (m)"; beam_offset "Offset (m)"; beam_color "Color (rgb)"; beam_opc "Opacity (0-1)"
      mask DialogControl Container4 Prompt: Beam
  Sensor : Subsystem
  F : PMIOPort  Side=Left
  Box : PMIOPort  Port=2  Side=Right
  p : Outport  VectorParamsAs1DForOutWhenUnconnected=off
  wires:
  Sensor/1(p) -> p/1
  connections:
  Geometry/RConn1 -- Sensor/LConn1 -- F/RConn1
  Box/RConn1 -- Sensor/RConn1

== system youBot_Arm_before_acceleration_test/Arm/Environment/Conveyors/Belt In/Normal Force ==
  bus : Inport
  Bus Selector3 : BusSelector  OutputSignals=fz1.Normal Force,fz2.Normal Force,fz3.Normal Force,fz4.Normal Force
  Sum : Sum  Inputs=++++
  sum : Outport  VectorParamsAs1DForOutWhenUnconnected=off
  wires:
  Bus Selector3/2 -> Sum/2  "<Normal Force>"
  Bus Selector3/4 -> Sum/4  "<Normal Force>"
  Bus Selector3/3 -> Sum/3  "<Normal Force>"
  Bus Selector3/1 -> Sum/1  "<Normal Force>"
  Sum/1 -> sum/1
  bus/1 -> Bus Selector3/1

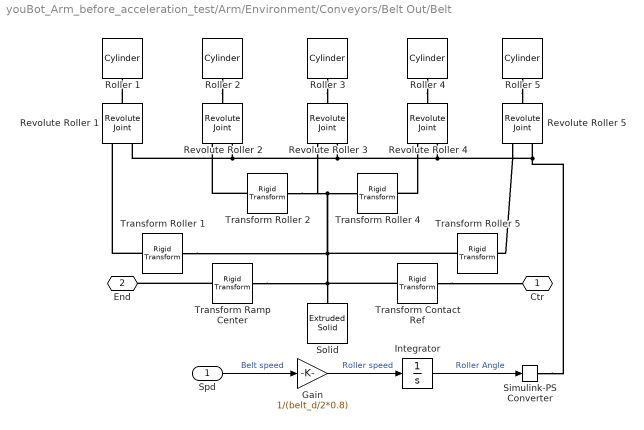
== system youBot_Arm_before_acceleration_test/Arm/Environment/Conveyors/Belt Out/Belt ==
  Spd : Inport
  Gain : Gain  Gain=1/(belt_d/2*0.8)
  Integrator : Integrator
  Revolute Roller {1..5} (5 alike) : sm_lib/Joints/Revolute Joint  JointMode=Normal  CompositeWrenchDir=FollowerOnBase  CompositeWrenchFrame=BaseFrame  SenseConstraintForce=off  SenseConstraintTorque=off  SenseTotalForce=off  SenseTotalTorque=off  PositionTargetSpecify=off  PositionTargetPriority=High  PositionTargetValue=0  PositionTargetValueUnits=deg  VelocityTargetSpecify=off  VelocityTargetPriority=High  VelocityTargetValue=0  VelocityTargetValueUnits=deg/s  EquilibriumPosition=0  EquilibriumPositionUnits=deg  SpringStiffness=0  SpringStiffnessUnits=N*m/deg  DampingCoefficient=0  DampingCoefficientUnits=N*m/(deg/s)  LowerLimitSpecify=off  LowerLimitBound=-90  LowerLimitBoundUnits=deg  LowerLimitStiffness=1e4  LowerLimitStiffnessUnits=N*m/deg  LowerLimitDamping=10  LowerLimitDampingUnits=N*m/(deg/s)  LowerLimitTransitionRegionWidth=0.1  LowerLimitTransitionRegionWidthUnits=deg  UpperLimitSpecify=off  UpperLimitBound=90  UpperLimitBoundUnits=deg  UpperLimitStiffness=1e4  UpperLimitStiffnessUnits=N*m/deg  UpperLimitDamping=10  UpperLimitDampingUnits=N*m/(deg/s)  UpperLimitTransitionRegionWidth=0.1  UpperLimitTransitionRegionWidthUnits=deg  TorqueActuationMode=ComputedTorque  MotionActuationMode=InputMotion  SensePosition=off  SenseVelocity=off  SenseAcceleration=off  SenseTorqueForce=off  SenseLowerLimitTorqueForce=off  SenseUpperLimitTorqueForce=off
  Roller {1..5} (5 alike) : Parts_Lib/Cylinder  Tag=CustomStyle  cyl_radius=belt_d/2*0.8  cyl_length=belt_w  cyl_density=1000  cyl_color=custom  cyl_opacity=1  cyl_color_custom=roller_clr  mark_radius=[0.75 0.5]  mark_len_factor=1.01  mark_angle=60  mark_color=black  mark_opacity=1
  Simulink-PS Converter : nesl_utility/Simulink-PS Converter  PhysicalDomain=network_engine_domain  SubClassName=ps_input  LeftPortType=input  RightPortType=output  PseudoPeriodic=off  Frequencies=[]  NoiseDistribution=none  NoiseParameters=[]  Unit=1  AffineConversion=off  FilteringAndDerivatives=filter  SimscapeFilterOrder=2  InputFilterTimeConstant=0.005  UdotUserProvided=1
  Solid : sm_lib/Body Elements/Extruded Solid  ExtrusionType=General  PolygonNumSides=3  PolygonOuterRadius=1  PolygonOuterRadiusUnits=m  ExportEntireGeometry=off  ExtrusionCrossSection=Extr_Data_LinkHoles(belt_l,belt_d,0.8*belt_d/2,5)  ExtrusionCrossSectionUnits=m  ExportConvexHullGeometry=off  ExtrusionLength=belt_w  ExtrusionLengthUnits=m  InertiaType=CalculateFromGeometry  BasedOnType=Density  Density=1000  DensityUnits=kg/(m^3)  Mass=1  MassUnits=kg  CenterOfMass=[0 0 0]  CenterOfMassUnits=m  MomentsOfInertia=[1 1 1]  MomentsOfInertiaUnits=kg*m^2  ProductsOfInertia=[0 0 0]  ProductsOfInertiaUnits=kg*m^2  GraphicType=FromGeometry  MarkerShape=Sphere  MarkerSize=10  GraphicVisPropType=SimpleVisualProperties  GraphicDiffuseColor=[0.5 0.5 0.5]  GraphicOpacity=1.0  GraphicSpecularColor=[0.5 0.5 0.5 1.0]  GraphicAmbientColor=[0.15 0.15 0.15 1.0]  GraphicEmissiveColor=[0.0 0.0 0.0 1.0]  GraphicShininess=75  DoExposeReferenceFrame=on  SerializedFrames=<Frames/>
  Transform Contact Ref : sm_lib/Frames and Transforms/Rigid Transform  RotationMethod=RotationSequence  FollAlignAxisA=+X  BaseAlignAxisA=+Y  FollAlignAxisB=+Y  BaseAlignAxisB=+Z  RotationStandardAxis=+Z  RotationAngle=0  RotationAngleUnits=deg  RotationArbitraryAxis=[0 0 1]  RotationSequenceAxes=FollowerAxes  RotationSequence=XYZ  RotationSequenceAngles=[-90 0 0]  RotationSequenceAnglesUnits=deg  RotationMatrix=[1 0 0; 0 1 0; 0 0 1]  Quaternion=[1 0 0 0]  TranslationMethod=None  TranslationCartesianOffset=[0 0 0]  TranslationCartesianOffsetUnits=m  TranslationStandardAxis=+X  TranslationStandardOffset=3/2  TranslationStandardOffsetUnits=m  TranslationROffset=0  TranslationROffsetUnits=m  TranslationThetaOffset=0  TranslationThetaOffsetUnits=deg  TranslationZOffset=0  TranslationZOffsetUnits=m
  Transform Ramp Center : sm_lib/Frames and Transforms/Rigid Transform  RotationMethod=None  FollAlignAxisA=+X  BaseAlignAxisA=+Y  FollAlignAxisB=+Y  BaseAlignAxisB=+Z  RotationStandardAxis=+Z  RotationAngle=0  RotationAngleUnits=deg  RotationArbitraryAxis=[0 0 1]  RotationSequenceAxes=FollowerAxes  RotationSequence=XYX  RotationSequenceAngles=[0 0 0]  RotationSequenceAnglesUnits=deg  RotationMatrix=[1 0 0; 0 1 0; 0 0 1]  Quaternion=[1 0 0 0]  TranslationMethod=StandardAxis  TranslationCartesianOffset=[0 0 0]  TranslationCartesianOffsetUnits=m  TranslationStandardAxis=+X  TranslationStandardOffset=belt_l/2  TranslationStandardOffsetUnits=m  TranslationROffset=0  TranslationROffsetUnits=m  TranslationThetaOffset=0  TranslationThetaOffsetUnits=deg  TranslationZOffset=0  TranslationZOffsetUnits=m
  Transform Roller 1 : sm_lib/Frames and Transforms/Rigid Transform  RotationMethod=None  FollAlignAxisA=+X  BaseAlignAxisA=+Y  FollAlignAxisB=+Y  BaseAlignAxisB=+Z  RotationStandardAxis=+Z  RotationAngle=0  RotationAngleUnits=deg  RotationArbitraryAxis=[0 0 1]  RotationSequenceAxes=FollowerAxes  RotationSequence=XYX  RotationSequenceAngles=[0 0 0]  RotationSequenceAnglesUnits=deg  RotationMatrix=[1 0 0; 0 1 0; 0 0 1]  Quaternion=[1 0 0 0]  TranslationMethod=StandardAxis  TranslationCartesianOffset=[0 0 0]  TranslationCartesianOffsetUnits=m  TranslationStandardAxis=-X  TranslationStandardOffset=belt_l/2  TranslationStandardOffsetUnits=m  TranslationROffset=0  TranslationROffsetUnits=m  TranslationThetaOffset=0  TranslationThetaOffsetUnits=deg  TranslationZOffset=0  TranslationZOffsetUnits=m
  Transform Roller 2 : sm_lib/Frames and Transforms/Rigid Transform  RotationMethod=None  FollAlignAxisA=+X  BaseAlignAxisA=+Y  FollAlignAxisB=+Y  BaseAlignAxisB=+Z  RotationStandardAxis=+Z  RotationAngle=0  RotationAngleUnits=deg  RotationArbitraryAxis=[0 0 1]  RotationSequenceAxes=FollowerAxes  RotationSequence=XYX  RotationSequenceAngles=[0 0 0]  RotationSequenceAnglesUnits=deg  RotationMatrix=[1 0 0; 0 1 0; 0 0 1]  Quaternion=[1 0 0 0]  TranslationMethod=StandardAxis  TranslationCartesianOffset=[0 0 0]  TranslationCartesianOffsetUnits=m  TranslationStandardAxis=-X  TranslationStandardOffset=belt_l/4  TranslationStandardOffsetUnits=m  TranslationROffset=0  TranslationROffsetUnits=m  TranslationThetaOffset=0  TranslationThetaOffsetUnits=deg  TranslationZOffset=0  TranslationZOffsetUnits=m
  Transform Roller 4 : sm_lib/Frames and Transforms/Rigid Transform  RotationMethod=None  FollAlignAxisA=+X  BaseAlignAxisA=+Y  FollAlignAxisB=+Y  BaseAlignAxisB=+Z  RotationStandardAxis=+Z  RotationAngle=0  RotationAngleUnits=deg  RotationArbitraryAxis=[0 0 1]  RotationSequenceAxes=FollowerAxes  RotationSequence=XYX  RotationSequenceAngles=[0 0 0]  RotationSequenceAnglesUnits=deg  RotationMatrix=[1 0 0; 0 1 0; 0 0 1]  Quaternion=[1 0 0 0]  TranslationMethod=StandardAxis  TranslationCartesianOffset=[0 0 0]  TranslationCartesianOffsetUnits=m  TranslationStandardAxis=+X  TranslationStandardOffset=belt_l/4  TranslationStandardOffsetUnits=m  TranslationROffset=0  TranslationROffsetUnits=m  TranslationThetaOffset=0  TranslationThetaOffsetUnits=deg  TranslationZOffset=0  TranslationZOffsetUnits=m
  Transform Roller 5 : sm_lib/Frames and Transforms/Rigid Transform  RotationMethod=None  FollAlignAxisA=+X  BaseAlignAxisA=+Y  FollAlignAxisB=+Y  BaseAlignAxisB=+Z  RotationStandardAxis=+Z  RotationAngle=0  RotationAngleUnits=deg  RotationArbitraryAxis=[0 0 1]  RotationSequenceAxes=FollowerAxes  RotationSequence=XYX  RotationSequenceAngles=[0 0 0]  RotationSequenceAnglesUnits=deg  RotationMatrix=[1 0 0; 0 1 0; 0 0 1]  Quaternion=[1 0 0 0]  TranslationMethod=StandardAxis  TranslationCartesianOffset=[0 0 0]  TranslationCartesianOffsetUnits=m  TranslationStandardAxis=+X  TranslationStandardOffset=belt_l/2  TranslationStandardOffsetUnits=m  TranslationROffset=0  TranslationROffsetUnits=m  TranslationThetaOffset=0  TranslationThetaOffsetUnits=deg  TranslationZOffset=0  TranslationZOffsetUnits=m
  Ctr : PMIOPort  Side=Right
  End : PMIOPort  Port=2  Side=Left
  wires:
  Integrator/1 -> Simulink-PS Converter/1  "Roller Angle"
  Gain/1 -> Integrator/1  "Roller speed"
  Spd/1 -> Gain/1  "Belt speed"
  connections:
  Revolute Roller 5/LConn2 -- Revolute Roller 4/LConn2 -- Revolute Roller 3/LConn2 -- Revolute Roller 2/LConn2 -- Revolute Roller 1/LConn2 -- Simulink-PS Converter/RConn1
  Roller 5/LConn1 -- Revolute Roller 5/RConn1
  Roller 4/LConn1 -- Revolute Roller 4/RConn1
  Roller 3/LConn1 -- Revolute Roller 3/RConn1
  Roller 2/LConn1 -- Revolute Roller 2/RConn1
  Transform Roller 1/RConn1 -- Revolute Roller 1/LConn1
  Revolute Roller 5/LConn1 -- Transform Roller 5/RConn1
  Revolute Roller 4/LConn1 -- Transform Roller 4/RConn1
  Transform Roller 2/RConn1 -- Revolute Roller 2/LConn1
  Revolute Roller 1/RConn1 -- Roller 1/LConn1
  Transform Ramp Center/LConn1 -- End/RConn1
  Transform Contact Ref/RConn1 -- Transform Ramp Center/RConn1 -- Transform Roller 5/LConn1 -- Transform Roller 1/LConn1 -- Transform Roller 4/LConn1 -- Transform Roller 2/LConn1 -- Revolute Roller 3/LConn1 -- Solid/RConn1
  Transform Contact Ref/LConn1 -- Ctr/RConn1

== system youBot_Arm_before_acceleration_test/Arm/Environment/Conveyors/Belt Out/Create Bus ==
  vx : Inport
  Bus Creator : BusCreator  Inputs=3
  Enable : Constant
  vy : Constant  Value=0
  bus : Outport  VectorParamsAs1DForOutWhenUnconnected=off
  wires:
  Bus Creator/1 -> bus/1
  vx/1 -> Bus Creator/2
  vy/1 -> Bus Creator/3  "vy"
  Enable/1 -> Bus Creator/1  "Enable"

== system youBot_Arm_before_acceleration_test/Arm/Environment/Conveyors/Belt Out/Detect Box ==
  Fn : Inport
  1/duration : Gain  Gain=1/dur_presence
  Check Weight : simulink/Logic and Bit Operations/Compare To Constant  relop=>=  const=box_weight  OutDataTypeStr=boolean  ZeroCross=off
  Compare To Zero : simulink/Logic and Bit Operations/Compare To Zero  relop=<=  OutDataTypeStr=boolean  ZeroCross=off
  Data Type Conversion : DataTypeConversion  OutDataTypeStr=double  SaturateOnIntegerOverflow=off  RndMeth=Floor
  Integrator : Integrator  ExternalReset=either
  Limit Level : Saturate  UpperLimit=box_weight  LowerLimit=0  ZeroCross=off
  Max Force : Saturate  UpperLimit=box_weight  LowerLimit=0
  Scope : Scope  NumInputPorts=2
  Unit Delay : UnitDelay  SampleTime=0.1  HasFrameUpgradeWarning=on
  On : Outport  VectorParamsAs1DForOutWhenUnconnected=off
  wires:
  Fn/1 -> Max Force/1
  Max Force/1 -> 1/duration/1
  Integrator/1 -> Limit Level/1
  Limit Level/1 -> Check Weight/1
  Compare To Zero/1 -> Integrator/2
  Check Weight/1 -> Data Type Conversion/1, Scope/2  "Enable Belt"
  Data Type Conversion/1 -> Unit Delay/1
  Unit Delay/1 -> On/1
  1/duration/1 -> Scope/1, Compare To Zero/1, Integrator/1

== system youBot_Arm_before_acceleration_test/Arm/Environment/Conveyors/Belt Out/Light Curtain ==
  Geometry : Subsystem  mask{beam_length=YBT_Par.BeltOut.Sensor.Beam.length, beam_radius=YBT_Par.BeltOut.Sensor.Beam.radius, beam_offset=YBT_Par.BeltOut.Sensor.Beam.offset, beam_color=YBT_Par.BeltOut.Sensor.Beam.color, beam_opc=YBT_Par.BeltOut.Sensor.Beam.opacity}
      mask prompts: beam_length "Length (m)"; beam_radius "Radius (m)"; beam_offset "Offset (m)"; beam_color "Color (rgb)"; beam_opc "Opacity (0-1)"
      mask DialogControl Container4 Prompt: Beam
  Sensor : Subsystem
  F : PMIOPort  Side=Left
  Box : PMIOPort  Port=2  Side=Right
  p : Outport  VectorParamsAs1DForOutWhenUnconnected=off
  wires:
  Sensor/1(p) -> p/1
  connections:
  Box/RConn1 -- Sensor/RConn1
  Sensor/LConn1 -- Geometry/RConn1 -- F/RConn1

== system youBot_Arm_before_acceleration_test/Arm/Environment/Conveyors/Belt Out/Normal Force ==
  bus : Inport
  Bus Selector3 : BusSelector  OutputSignals=fz1.Normal Force,fz2.Normal Force,fz3.Normal Force,fz4.Normal Force
  Sum : Sum  Inputs=++++
  sum : Outport  VectorParamsAs1DForOutWhenUnconnected=off
  wires:
  Bus Selector3/2 -> Sum/2  "<Normal Force>"
  Bus Selector3/4 -> Sum/4  "<Normal Force>"
  Bus Selector3/3 -> Sum/3  "<Normal Force>"
  Bus Selector3/1 -> Sum/1  "<Normal Force>"
  Sum/1 -> sum/1
  bus/1 -> Bus Selector3/1
